simulink subsystem "Slosh"  (R2026a)
settings: Solver=VariableStepAuto
undefined symbols (not defined in the file): fu_axial_damping_ratios, fu_lateral_damping_ratios, fu_mass_profile, IN, ox_axial_damping_ratios, ox_lateral_damping_ratios, ox_mass_profile
libraries: matrix_library x8
settings Model: Creator=asing  LastModifiedBy=asing

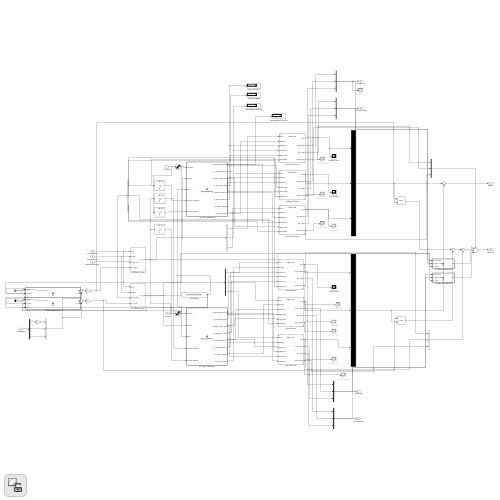
[thumbnail: Simulink's stored preview of the top-level diagram]
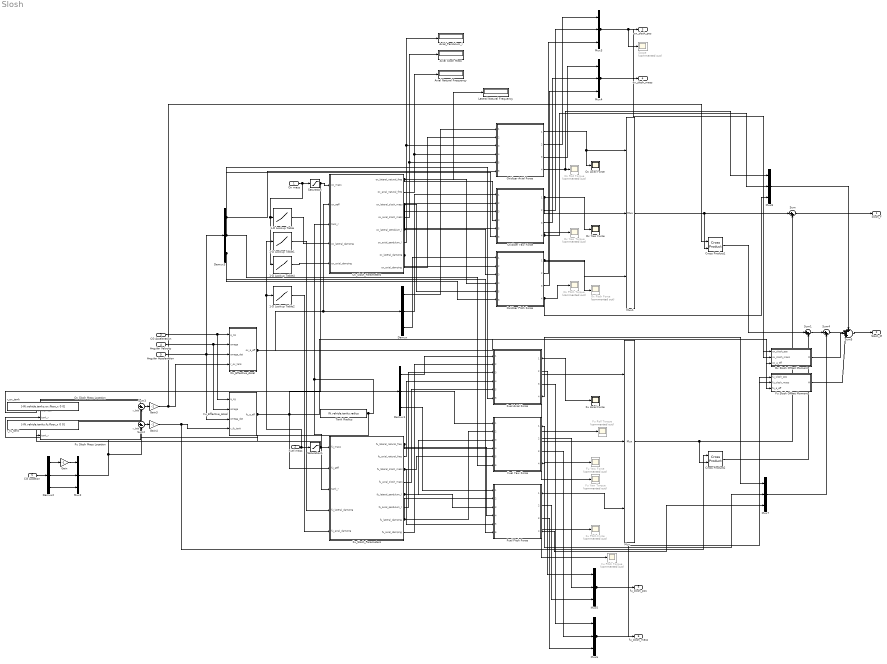
== system Slosh ==
  Ox mass : Inport
  Fuel mass : Inport  Port=2
  CG Acceleration : Inport  Port=3
  Angular Velocity : Inport  Port=4
  Angular Acceleration : Inport  Port=5
  CG Location : Inport  Port=6
  1-D Lookup Table : Lookup_n-D  NumberOfTableDimensions=1  BreakpointsForDimension1=ox_mass_profile  Table=ox_lateral_damping_ratios  InternalRulePriority=Speed  RndMeth=Simplest
  1-D Lookup Table1 : Lookup_n-D  NumberOfTableDimensions=1  BreakpointsForDimension1=fu_mass_profile  Table=fu_lateral_damping_ratios  InternalRulePriority=Speed  RndMeth=Simplest
  1-D Lookup Table2 : Lookup_n-D  NumberOfTableDimensions=1  BreakpointsForDimension1=fu_mass_profile  Table=fu_axial_damping_ratios  InternalRulePriority=Speed  RndMeth=Simplest
  1-D Lookup Table4 : Lookup_n-D  NumberOfTableDimensions=1  BreakpointsForDimension1=ox_mass_profile  Table=ox_axial_damping_ratios  InternalRulePriority=Speed  RndMeth=Simplest
  Axial Natural Frequency : Display
  Axial Slosh Mass : Display
  Axial_Pendulum_l : Display
  Cross Product1 : matrix_library/Cross Product
  Cross Product2 : matrix_library/Cross Product
  Demux{,1..3} (4 alike) : Demux  Outputs=3
  Fu Axial Force : Scope
      settings: ActiveDisplayYMinimum=-4.5487995330933861  ActiveDisplayYMaximum=10.430303988696288  DataLoggingVariableName=ScopeData38
  Fu Pitch Force : Scope  Commented=on
      settings: ActiveDisplayYMinimum=-2.9742058993087932  ActiveDisplayYMaximum=15.331760127930639  DataLoggingVariableName=ScopeData40
  Fu Pitch Torque : Scope  Commented=on
      settings: ActiveDisplayYMinimum=-0.19116574787256713  ActiveDisplayYMaximum=0.19970427620804132  DataLoggingVariableName=ScopeData87
  Fu Roll Torque : Scope  Commented=on
      settings: ActiveDisplayYMinimum=-9.5580450498277436  ActiveDisplayYMaximum=8.6061310713641461  DataLoggingVariableName=ScopeData86
  Fu Slosh Mass Location : MATLAB Function  TreatAsAtomicUnit=on
  Fu Slosh Offset Moment : MATLAB Function  TreatAsAtomicUnit=on
  Fu Yaw Force : Scope  Commented=on
      settings: ActiveDisplayYMinimum=-1.96682346554972  ActiveDisplayYMaximum=2.7427386100438831  DataLoggingVariableName=ScopeData39
  Fu Yaw Torque : Scope  Commented=on
      settings: ActiveDisplayYMinimum=-3.6886267521568623  ActiveDisplayYMaximum=3.9647425854021145  DataLoggingVariableName=ScopeData82
  Fu_Effective_Accel : Subsystem
  Fu_Slosh_Parameters : MATLAB Function  TreatAsAtomicUnit=on
  Fuel Axial Force : Subsystem  ReferencedSubsystem=Slosh_Axis
  Fuel Pitch Force : Subsystem  ReferencedSubsystem=Slosh_Axis
  Fuel Yaw Force : Subsystem  ReferencedSubsystem=Slosh_Axis
  Gain : Gain  Gain=-1
  Gain3 : Gain  Gain=-1
  Gain4 : Gain  Gain=-1
  Lateral Natural Frequency : Display
  Mux{,1..8} (9 alike) : Mux  Inputs=3
  Ox Axial Force : Scope
      settings: ActiveDisplayYMinimum=-3.9644122254155478  ActiveDisplayYMaximum=18.110904773524471  DataLoggingVariableName=ScopeData34
  Ox Pitch Force : Scope  Commented=on
      settings: ActiveDisplayYMinimum=-4.4950785008236629  ActiveDisplayYMaximum=22.001881619828325  DataLoggingVariableName=ScopeData36
  Ox Pitch Torque : Scope  Commented=on
      settings: ActiveDisplayYMinimum=-0.69593653498138675  ActiveDisplayYMaximum=0.79680864639954685  DataLoggingVariableName=ScopeData85
  Ox Roll Torque : Scope  Commented=on
      settings: ActiveDisplayYMinimum=-0.15656949128956149  ActiveDisplayYMaximum=0.79158034254760723  DataLoggingVariableName=ScopeData80
  Ox Slosh Mass Location : MATLAB Function  TreatAsAtomicUnit=on
  Ox Slosh Offset Moment : MATLAB Function  TreatAsAtomicUnit=on
  Ox Yaw Force : Scope
      settings: ActiveDisplayYMinimum=-5.8284827308381395  ActiveDisplayYMaximum=24.723450598791928  DataLoggingVariableName=ScopeData37
  Ox Yaw Torque : Scope  Commented=on
      settings: ActiveDisplayYMinimum=-0.3482323750211066  ActiveDisplayYMaximum=0.31743853430357161  DataLoggingVariableName=ScopeData81
  Ox_Effective_Accel : Subsystem
  Ox_Slosh_Parameters : MATLAB Function  TreatAsAtomicUnit=on
  Oxidizer Axial Force : Subsystem  ReferencedSubsystem=Slosh_Axis
  Oxidizer Pitch Force : Subsystem  ReferencedSubsystem=Slosh_Axis
  Oxidizer Yaw Force : Subsystem  ReferencedSubsystem=Slosh_Axis
  Saturation : Saturate  UpperLimit=inf  LowerLimit=0.01
  Saturation1 : Saturate  UpperLimit=inf  LowerLimit=0.01
  Scope : Scope  Commented=on
      settings: ActiveDisplayYMinimum=-0.0849364779794028  ActiveDisplayYMaximum=0.368207880424993  DataLoggingVariableName=ScopeData35
  Sum : Sum  Inputs=|++
  Sum1 : Sum  Inputs=|++
  Sum2 : Sum  Inputs=|+-
  Sum3 : Sum  Inputs=|+-
  Sum4 : Sum  Inputs=|++
  Sum5 : Sum  Inputs=++++|
  Tank Radius : Constant  Value=IN.vehicle.tanks.radius  SampleTime=-1
  r_fu_tank : Constant  Value=[-IN.vehicle.tanks.fu.floor_x 0 0]
  r_ox_tank : Constant  Value=[-IN.vehicle.tanks.ox.floor_x 0 0]
  Slosh_F : Outport
  Slosh_M : Outport  Port=2
  ox_slosh_pos : Outport  Port=3
  ox_slosh_mass : Outport  Port=4
  fu_slosh_pos : Outport  Port=5
  fu_slosh_mass : Outport  Port=6
  wires:
  Ox mass/1 -> Saturation/1, 1-D Lookup Table/1, 1-D Lookup Table4/1
  CG Acceleration/1 -> Fu_Effective_Accel/1(a_cg), Ox_Effective_Accel/1(a_cg)
  Angular Velocity/1 -> Fu_Effective_Accel/2(omega), Ox_Effective_Accel/2(omega)
  Angular Acceleration/1 -> Demux3/1, Fu_Effective_Accel/3(omega_dot), Ox_Effective_Accel/3(omega_dot)
  Fuel mass/1 -> Saturation1/1, 1-D Lookup Table1/1, 1-D Lookup Table2/1
  Ox_Effective_Accel/1(ox_a_eff) -> Ox Slosh Offset Moment/3(ox_a_eff), Ox_Slosh_Parameters/2(ox_aeff), Demux/1
  Fu_Effective_Accel/1(fu_a_eff) -> Fu Slosh Offset Moment/3(fu_a_eff), Fu_Slosh_Parameters/2(fu_aeff), Demux1/1
  Demux/1 -> Oxidizer Axial Force/1
  Ox_Slosh_Parameters/1(ox_lateral_natural_freq) -> Oxidizer Yaw Force/4, Lateral Natural Frequency/1, Oxidizer Pitch Force/4
  Ox_Slosh_Parameters/2(ox_axial_natural_freq) -> Oxidizer Axial Force/4, Axial Natural Frequency/1
  Ox_Slosh_Parameters/3(ox_lateral_slosh_mass) -> Oxidizer Yaw Force/5, Oxidizer Pitch Force/5
  Ox_Slosh_Parameters/4(ox_axial_slosh_mass) -> Oxidizer Axial Force/5, Axial Slosh Mass/1
  Ox_Slosh_Parameters/5(ox_lateral_pendulum_l) -> Oxidizer Yaw Force/3, Oxidizer Pitch Force/3
  Ox_Slosh_Parameters/6(ox_axial_pendulum_l) -> Oxidizer Axial Force/3, Axial_Pendulum_l/1
  Ox_Slosh_Parameters/7(ox_lateral_damping) -> Oxidizer Yaw Force/2, Oxidizer Pitch Force/2
  Ox_Slosh_Parameters/8(ox_axial_damping) -> Oxidizer Axial Force/2
  Fu_Slosh_Parameters/1(fu_lateral_natural_freq) -> Fuel Yaw Force/4, Fuel Pitch Force/4
  Fu_Slosh_Parameters/3(fu_lateral_slosh_mass) -> Fuel Yaw Force/5, Fuel Pitch Force/5
  Fu_Slosh_Parameters/5(fu_lateral_pendulum_l) -> Fuel Yaw Force/3, Fuel Pitch Force/3
  Fu_Slosh_Parameters/7(fu_lateral_damping) -> Fuel Yaw Force/2, Fuel Pitch Force/2
  Oxidizer Axial Force/1 -> Mux1/1, Ox Axial Force/1
  Mux1/1 -> Sum/1, Cross Product1/2
  Mux/1 -> Cross Product2/2, Sum/2
  Sum/1 -> Slosh_F/1
  Cross Product1/1 -> Sum1/1
  Cross Product2/1 -> Sum1/2
  Tank Radius/1 -> Fu Slosh Mass Location/3(tank_r), Ox Slosh Mass Location/3(tank_r), Ox_Slosh_Parameters/3(tank_r), Fu_Slosh_Parameters/3(tank_r)
  Mux2/1 -> Sum3/2, Sum2/2
  Sum3/1 -> Gain3/1
  Sum2/1 -> Gain4/1
  Gain3/1 -> Ox_Effective_Accel/4(r_ox_tank), Cross Product1/1
  Gain4/1 -> Fu_Effective_Accel/4(r_fu_tank), Cross Product2/1
  Demux2/3 -> Mux2/3
  CG Location/1 -> Demux2/1
  Demux2/2 -> Mux2/2
  Demux2/1 -> Gain/1
  Gain/1 -> Mux2/1
  Mux3/1 -> Ox Slosh Offset Moment/1(ox_slosh_pos), ox_slosh_pos/1, Scope/1
  Oxidizer Axial Force/3 -> Mux4/1
  Mux4/1 -> Ox Slosh Offset Moment/2(ox_slosh_mass), ox_slosh_mass/1
  Mux5/1 -> Fu Slosh Offset Moment/1(fu_slosh_pos), fu_slosh_pos/1
  Mux6/1 -> Fu Slosh Offset Moment/2(fu_slosh_mass), fu_slosh_mass/1
  Oxidizer Axial Force/2 -> Mux3/1
  Demux3/1 -> Fuel Axial Force/6, Oxidizer Axial Force/6
  Demux3/2 -> Fuel Yaw Force/6, Oxidizer Yaw Force/6
  Demux3/3 -> Fuel Pitch Force/6, Oxidizer Pitch Force/6
  Oxidizer Axial Force/4 -> Ox Roll Torque/1, Mux8/1
  Sum1/1 -> Sum4/1
  Sum5/1 -> Slosh_M/1
  Sum4/1 -> Sum5/2
  Mux8/1 -> Sum5/1
  Mux7/1 -> Sum4/2
  Saturation/1 -> Ox Slosh Mass Location/2(ox_mass), Ox_Slosh_Parameters/1(ox_mass)
  Saturation1/1 -> Fu Slosh Mass Location/2(fu_mass), Fu_Slosh_Parameters/1(fu_mass)
  1-D Lookup Table/1 -> Ox_Slosh_Parameters/4("ox_lateral_damping ")
  1-D Lookup Table1/1 -> Fu_Slosh_Parameters/4("fu_lateral_damping ")
  1-D Lookup Table4/1 -> Ox_Slosh_Parameters/5("ox_axial_damping ")
  1-D Lookup Table2/1 -> Fu_Slosh_Parameters/5("fu_axial_damping ")
  r_ox_tank/1 -> Ox Slosh Mass Location/1(r_floor)
  Ox Slosh Mass Location/1(r_bob) -> Sum3/1
  r_fu_tank/1 -> Fu Slosh Mass Location/1(r_floor)
  Fu Slosh Mass Location/1(r_bob) -> Sum2/1
  Ox Slosh Offset Moment/1(M) -> Sum5/3
  Fu Slosh Offset Moment/1(M) -> Sum5/4
  Demux/3 -> Oxidizer Pitch Force/1
  Oxidizer Pitch Force/1 -> Ox Pitch Force/1, Mux1/3
  Oxidizer Pitch Force/2 -> Mux3/3
  Oxidizer Pitch Force/3 -> Mux4/3
  Oxidizer Pitch Force/4 -> Mux8/3, Ox Pitch Torque/1
  Demux/2 -> Oxidizer Yaw Force/1
  Oxidizer Yaw Force/1 -> Mux1/2, Ox Yaw Force/1
  Oxidizer Yaw Force/2 -> Mux3/2
  Oxidizer Yaw Force/3 -> Mux4/2
  Oxidizer Yaw Force/4 -> Ox Yaw Torque/1, Mux8/2
  Demux1/1 -> Fuel Axial Force/1
  Fu_Slosh_Parameters/8(fu_axial_damping) -> Fuel Axial Force/2
  Fu_Slosh_Parameters/6(fu_axial_pendulum_l) -> Fuel Axial Force/3
  Fu_Slosh_Parameters/2(fu_axial_natural_freq) -> Fuel Axial Force/4
  Fu_Slosh_Parameters/4(fu_axial_slosh_mass) -> Fuel Axial Force/5
  Fuel Axial Force/1 -> Mux/1, Fu Axial Force/1
  Fuel Axial Force/2 -> Mux5/1
  Fuel Axial Force/3 -> Mux6/1
  Fuel Axial Force/4 -> Fu Roll Torque/1, Mux7/1
  Demux1/3 -> Fuel Pitch Force/1
  Fuel Pitch Force/1 -> Fu Pitch Force/1, Mux/3
  Fuel Pitch Force/2 -> Mux5/3
  Fuel Pitch Force/3 -> Mux6/3
  Fuel Pitch Force/4 -> Fu Pitch Torque/1, Mux7/3
  Demux1/2 -> Fuel Yaw Force/1
  Fuel Yaw Force/1 -> Mux/2, Fu Yaw Force/1
  Fuel Yaw Force/2 -> Mux5/2
  Fuel Yaw Force/3 -> Mux6/2
  Fuel Yaw Force/4 -> Fu Yaw Torque/1, Mux7/2

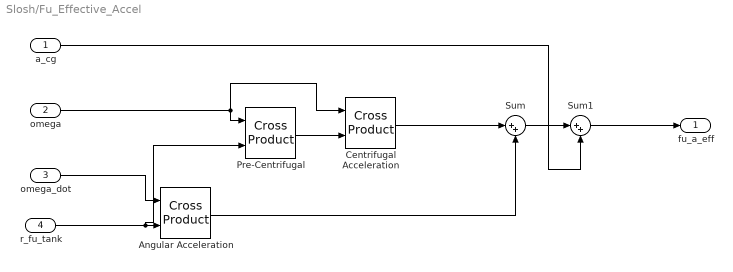
== system Slosh/Fu_Effective_Accel ==
  a_cg : Inport
  omega : Inport  Port=2
  omega_dot : Inport  Port=3
  r_fu_tank : Inport  Port=4
  Angular Acceleration : matrix_library/Cross Product
  Centrifugal Acceleration : matrix_library/Cross Product
  Pre-Centrifugal : matrix_library/Cross Product
  Sum : Sum  Inputs=|++
  Sum1 : Sum  Inputs=|++
  fu_a_eff : Outport
  wires:
  Sum1/1 -> fu_a_eff/1
  a_cg/1 -> Sum1/2
  Sum/1 -> Sum1/1
  Angular Acceleration/1 -> Sum/2
  Centrifugal Acceleration/1 -> Sum/1
  Pre-Centrifugal/1 -> Centrifugal Acceleration/2
  omega/1 -> Pre-Centrifugal/1, Centrifugal Acceleration/1
  omega_dot/1 -> Angular Acceleration/1
  r_fu_tank/1 -> Angular Acceleration/2, Pre-Centrifugal/2

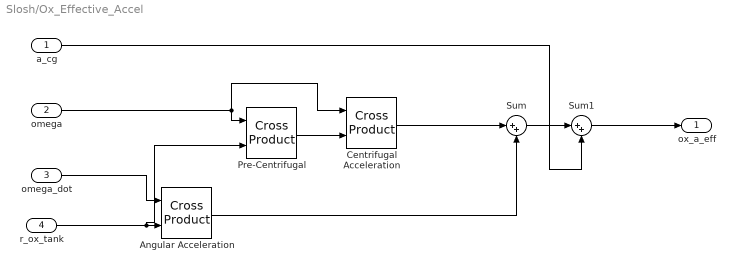
== system Slosh/Ox_Effective_Accel ==
  a_cg : Inport
  omega : Inport  Port=2
  omega_dot : Inport  Port=3
  r_ox_tank : Inport  Port=4
  Angular Acceleration : matrix_library/Cross Product
  Centrifugal Acceleration : matrix_library/Cross Product
  Pre-Centrifugal : matrix_library/Cross Product
  Sum : Sum  Inputs=|++
  Sum1 : Sum  Inputs=|++
  ox_a_eff : Outport
  wires:
  Sum1/1 -> ox_a_eff/1
  a_cg/1 -> Sum1/2
  Sum/1 -> Sum1/1
  Angular Acceleration/1 -> Sum/2
  Centrifugal Acceleration/1 -> Sum/1
  Pre-Centrifugal/1 -> Centrifugal Acceleration/2
  omega/1 -> Pre-Centrifugal/1, Centrifugal Acceleration/1
  omega_dot/1 -> Angular Acceleration/1
  r_ox_tank/1 -> Angular Acceleration/2, Pre-Centrifugal/2

== matlab function Slosh/Ox_Slosh_Parameters ==
  data: ox_lateral_natural_freq output; ox_axial_natural_freq output; ox_mass input; ox_lateral_slosh_mass output; ox_axial_slosh_mass output; ox_lateral_pendulum_l output; ox_aeff input; ox_axial_pendulum_l output; ox_lateral_damping output; ox_axial_damping output; tank_r input; ox_lateral_damping input; ox_axial_damping input
function [ox_lateral_natural_freq, ox_axial_natural_freq, ox_lateral_slosh_mass,ox_axial_slosh_mass, ox_lateral_pendulum_l, ox_axial_pendulum_l, ox_lateral_damping, ox_axial_damping]  = slosh_parameters(ox_mass, ox_aeff, tank_r, ox_lateral_damping, ox_axial_damping)

% Flat-bottomed cylindrical tank, linear slosh (NASA SP-106 / Dodge 2000;
% lateral values checked against SLOSH-ML, lgst-lab/slosh_ml).
zeta = 1.841;    % 1st root of J1' (1st lateral mode)
eps01 = 3.8317;  % 1st root of J1 (1st axisymmetric mode)
ox_density = 1141;   % kg/m^3
geff = norm(ox_aeff) + 0.001;

if ox_mass > 0.001
   h_ox_fluid = (ox_mass / ox_density) / (pi * tank_r^2);

   % Lateral mode: omega^2 = (g*xi/R) * tanh(xi*h/R)
    ox_lateral_natural_freq = sqrt(zeta * geff / tank_r * tanh(zeta * h_ox_fluid / tank_r));
    ox_lateral_slosh_mass = ox_mass * (2 * tank_r * tanh(zeta * h_ox_fluid / tank_r)) / (zeta * (zeta^2 - 1) * h_ox_fluid);
    ox_lateral_pendulum_l = tank_r / (zeta * tanh(zeta * h_ox_fluid / tank_r));   % = geff / omega^2

    % Axisymmetric (m = 0) mode: omega^2 = (g*eps01/R) * tanh(eps01*h/R).
    % Volume is conserved and the mode is axisymmetric, so to first order
    % it puts no net force or moment on the tank: its equivalent mechanical
    % mass is zero. The oscillator is kept (frequency/damping) but couples
    % no force or roll torque into the vehicle.
    ox_axial_natural_freq = sqrt(eps01 * geff / tank_r * tanh(eps01 * h_ox_fluid / tank_r));
    ox_axial_slosh_mass = 0;
    ox_axial_pendulum_l = geff / ox_axial_natural_freq^2;
else
   h_ox_fluid = 0;
   ox_lateral_natural_freq = 0;
   ox_axial_natural_freq = 0;
   ox_lateral_slosh_mass = 0;
   ox_axial_slosh_mass = 0;
   ox_lateral_pendulum_l = 1;
   ox_axial_pendulum_l = 1;
end

end

== matlab function Slosh/Fu_Slosh_Parameters ==
  data: fu_mass input; fu_lateral_natural_freq output; fu_axial_natural_freq output; fu_lateral_slosh_mass output; fu_aeff input; fu_axial_slosh_mass output; fu_lateral_pendulum_l output; fu_axial_pendulum_l output; fu_lateral_damping output; fu_axial_damping output; tank_r input; fu_lateral_damping input; fu_axial_damping input
function [fu_lateral_natural_freq, fu_axial_natural_freq, fu_lateral_slosh_mass,fu_axial_slosh_mass, fu_lateral_pendulum_l, fu_axial_pendulum_l, fu_lateral_damping, fu_axial_damping]  = slosh_parameters(fu_mass, fu_aeff, tank_r, fu_lateral_damping, fu_axial_damping)

% Flat-bottomed cylindrical tank, linear slosh (NASA SP-106 / Dodge 2000;
% lateral values checked against SLOSH-ML, lgst-lab/slosh_ml).
zeta = 1.841;    % 1st root of J1' (1st lateral mode)
eps01 = 3.8317;  % 1st root of J1 (1st axisymmetric mode)
fu_density = 800;   % kg/m^3
geff = norm(fu_aeff) + 0.001;

if fu_mass > 0.001
   h_fu_fluid = (fu_mass / fu_density) / (pi * tank_r^2);

   % Lateral mode: omega^2 = (g*xi/R) * tanh(xi*h/R)
    fu_lateral_natural_freq = sqrt(zeta * geff / tank_r * tanh(zeta * h_fu_fluid / tank_r));
    fu_lateral_slosh_mass = fu_mass * (2 * tank_r * tanh(zeta * h_fu_fluid / tank_r)) / (zeta * (zeta^2 - 1) * h_fu_fluid);
    fu_lateral_pendulum_l = tank_r / (zeta * tanh(zeta * h_fu_fluid / tank_r));   % = geff / omega^2

    % Axisymmetric (m = 0) mode: omega^2 = (g*eps01/R) * tanh(eps01*h/R).
    % Volume is conserved and the mode is axisymmetric, so to first order
    % it puts no net force or moment on the tank: its equivalent mechanical
    % mass is zero. The oscillator is kept (frequency/damping) but couples
    % no force or roll torque into the vehicle.
    fu_axial_natural_freq = sqrt(eps01 * geff / tank_r * tanh(eps01 * h_fu_fluid / tank_r));
    fu_axial_slosh_mass = 0;
    fu_axial_pendulum_l = geff / fu_axial_natural_freq^2;
else
   h_fu_fluid = 0;
   fu_lateral_natural_freq = 0;
   fu_axial_natural_freq = 0;
   fu_lateral_slosh_mass = 0;
   fu_axial_slosh_mass = 0;
   fu_lateral_pendulum_l = 1;
   fu_axial_pendulum_l = 1;
end

end

== matlab function Slosh/Ox Slosh Mass Location ==
  data: r_floor input; r_bob output; ox_mass input; tank_r input
function r_bob = fcn(r_floor, ox_mass, tank_r)
% Rest position of the 1st lateral pendulum bob (= spring-mass location),
% flat-bottom cylinder, NASA SP-106 / Dodge 2000:
%   H1 = h - (2R/xi) tanh(xi h / 2R)  above the tank floor,
%   hinge = H1 + L1,  L1 = R / (xi tanh(xi h / R)).
% Matches SLOSH-ML (validation/slosh_ml/compareSloshML.m) to < 2 mm.
% The slosh force is applied here, not at the hinge: the propellant
% (bob included) is already a rigid body in the CG/MOI tables, so the
% pendulum correction is -m1*y_ddot at the bob rest point plus the
% offset moment -m1*y x f (Slosh offset moment blocks); together these
% equal the rod force acting at the hinge.
% r_floor is in the Slosh frame (datum x negated).
xi = 1.841;
ox_density = 1141;   % kg/m^3
h = (ox_mass / ox_density) / (pi * tank_r^2);
H1 = h - (2 * tank_r / xi) * tanh(xi * h / (2 * tank_r));
r_bob = r_floor;
r_bob(1) = r_floor(1) - H1;

== matlab function Slosh/Fu Slosh Mass Location ==
  data: r_floor input; r_bob output; fu_mass input; tank_r input
function r_bob = fcn(r_floor, fu_mass, tank_r)
% Rest position of the 1st lateral pendulum bob (= spring-mass location),
% flat-bottom cylinder, NASA SP-106 / Dodge 2000:
%   H1 = h - (2R/xi) tanh(xi h / 2R)  above the tank floor,
%   hinge = H1 + L1,  L1 = R / (xi tanh(xi h / R)).
% Matches SLOSH-ML (validation/slosh_ml/compareSloshML.m) to < 2 mm.
% The slosh force is applied here, not at the hinge: the propellant
% (bob included) is already a rigid body in the CG/MOI tables, so the
% pendulum correction is -m1*y_ddot at the bob rest point plus the
% offset moment -m1*y x f (Slosh offset moment blocks); together these
% equal the rod force acting at the hinge.
% r_floor is in the Slosh frame (datum x negated).
xi = 1.841;
fu_density = 800;   % kg/m^3
h = (fu_mass / fu_density) / (pi * tank_r^2);
H1 = h - (2 * tank_r / xi) * tanh(xi * h / (2 * tank_r));
r_bob = r_floor;
r_bob(1) = r_floor(1) - H1;

== matlab function Slosh/Ox Slosh Offset Moment ==
  data: ox_slosh_pos input; M output; ox_slosh_mass input; ox_a_eff input
function M = fcn(ox_slosh_pos, ox_slosh_mass, ox_a_eff)
% Moment about the CG from the slosh mass displaced by y from its rest
% point, under the specific force f at the tank: -m1 * y x f. With the
% -m1*y_ddot force at the rest point this is the first-order pendulum
% load (rod force at the hinge). Replaces the slosh CG shift in
% CG // MOI Script v3, which divided by the propellant mass instead of
% the vehicle mass, had the lateral sign reversed, and was delayed.
M = reshape(-cross(ox_slosh_mass(:) .* ox_slosh_pos(:), ox_a_eff(:)), size(ox_a_eff));

== matlab function Slosh/Fu Slosh Offset Moment ==
  data: fu_slosh_pos input; M output; fu_slosh_mass input; fu_a_eff input
function M = fcn(fu_slosh_pos, fu_slosh_mass, fu_a_eff)
% Moment about the CG from the slosh mass displaced by y from its rest
% point, under the specific force f at the tank: -m1 * y x f. With the
% -m1*y_ddot force at the rest point this is the first-order pendulum
% load (rod force at the hinge). Replaces the slosh CG shift in
% CG // MOI Script v3, which divided by the propellant mass instead of
% the vehicle mass, had the lateral sign reversed, and was delayed.
M = reshape(-cross(fu_slosh_mass(:) .* fu_slosh_pos(:), fu_a_eff(:)), size(fu_a_eff));
